simulink model "kalman_position_velocity"  (R2025b)
settings: Solver=FixedStepDiscrete  StartTime=0.0  StopTime=20  FixedStep=0.1  RelTol=1e-3
settings Model: Creator=alosw  LastModifiedBy=alosw

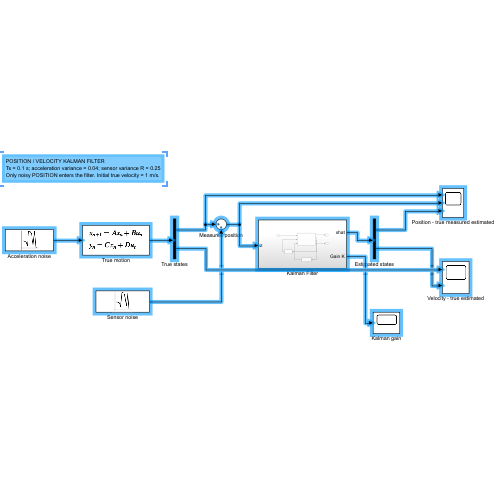
[thumbnail: Simulink's stored preview of the top-level diagram]
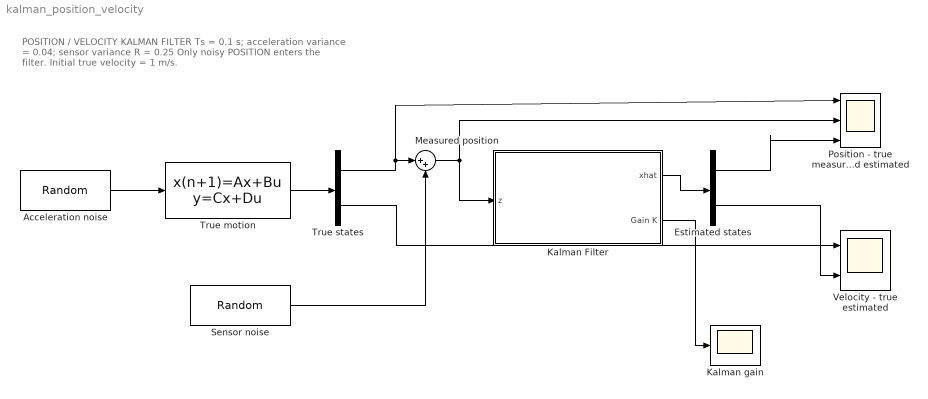
== system kalman_position_velocity ==
  note: POSITION / VELOCITY KALMAN FILTER
      | Ts = 0.1 s; acceleration variance = 0.04; sensor variance R = 0.25
      | Only noisy POSITION enters the filter. Initial true velocity = 1 m/s.
  Acceleration noise : RandomNumber  Variance=0.04  Seed=1234  SampleTime=0.1
  Estimated states : Demux  Outputs=2
  Kalman Filter : Subsystem
  Kalman gain : Scope
  Measured position : Sum  Inputs=|++
  Position - true measured estimated : Scope  NumInputPorts=3
  Sensor noise : RandomNumber  Variance=0.25  Seed=5678  SampleTime=0.1
  True motion : DiscreteStateSpace  A=[1 0.1;0 1]  B=[0.005;0.1]  C=eye(2)  D=zeros(2,1)  InitialCondition=[0;1]  SampleTime=0.1
  True states : Demux  Outputs=2
  Velocity - true estimated : Scope  NumInputPorts=2
  wires:
  Acceleration noise/1 -> True motion/1
  True motion/1 -> True states/1
  True states/1 -> Position - true measured estimated/1, Measured position/1
  Sensor noise/1 -> Measured position/2
  Measured position/1 -> Position - true measured estimated/2, Kalman Filter/1(z)
  Kalman Filter/1(xhat) -> Estimated states/1
  Estimated states/1 -> Position - true measured estimated/3
  True states/2 -> Velocity - true estimated/1
  Estimated states/2 -> Velocity - true estimated/2
  Kalman Filter/2(Gain K) -> Kalman gain/1

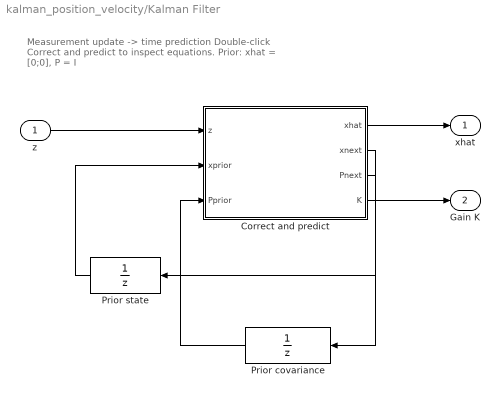
== system kalman_position_velocity/Kalman Filter ==
  note: Measurement update -> time prediction
      | Double-click Correct and predict to inspect equations.
      | Prior: xhat = [0;0], P = I
  z : Inport
  Correct and predict : MATLAB Function  TreatAsAtomicUnit=on
  Prior covariance : UnitDelay  InitialCondition=eye(2)  SampleTime=0.1  HasFrameUpgradeWarning=on
  Prior state : UnitDelay  InitialCondition=[0;0]  SampleTime=0.1  HasFrameUpgradeWarning=on
  xhat : Outport
  Gain K : Outport  Port=2
  wires:
  z/1 -> Correct and predict/1(z)
  Prior state/1 -> Correct and predict/2(xprior)
  Prior covariance/1 -> Correct and predict/3(Pprior)
  Correct and predict/1(xhat) -> xhat/1
  Correct and predict/2(xnext) -> Prior state/1
  Correct and predict/3(Pnext) -> Prior covariance/1
  Correct and predict/4(K) -> Gain K/1

== matlab function kalman_position_velocity/Kalman Filter/Correct and predict ==
  data: z input; xhat output; xprior input; Pprior input; xnext output; Pnext output; K output
function [xhat,xnext,Pnext,K] = kf_step(z,xprior,Pprior)
%#codegen
% Correct the current prior, then predict the next sample.
Ts = 0.1;
A = [1 Ts; 0 1];
H = [1 0];
G = [Ts^2/2; Ts];
Q = 0.04*(G*G');
R = 0.25;
K = Pprior*H'/(H*Pprior*H'+R);
xhat = xprior + K*(z-H*xprior);
J = eye(2)-K*H;
Ppost = J*Pprior*J' + K*R*K';
xnext = A*xhat;
Pnext = A*Ppost*A'+Q;
Pnext = (Pnext+Pnext')/2;
end
